simulink model "L150_Auto_Segments"  (R2026a)
settings: Solver=VariableStepAuto  StopTime=40.0
undefined symbols (not defined in the file): routeData, routeDirs, stopState
libraries: robotmobilelib x1, simulink x1
settings Model: Creator=hanjiatong  LastModifiedBy=hanjiatong

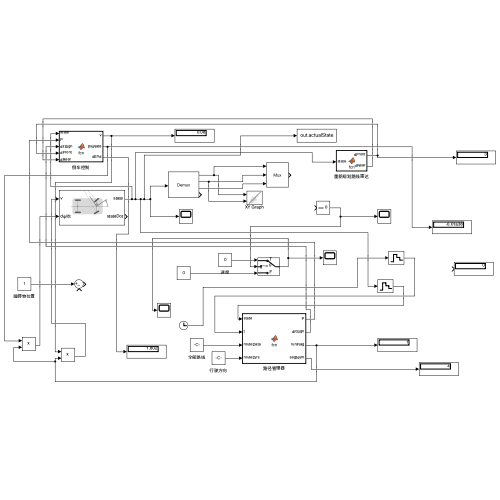
[thumbnail: Simulink's stored preview of the top-level diagram]
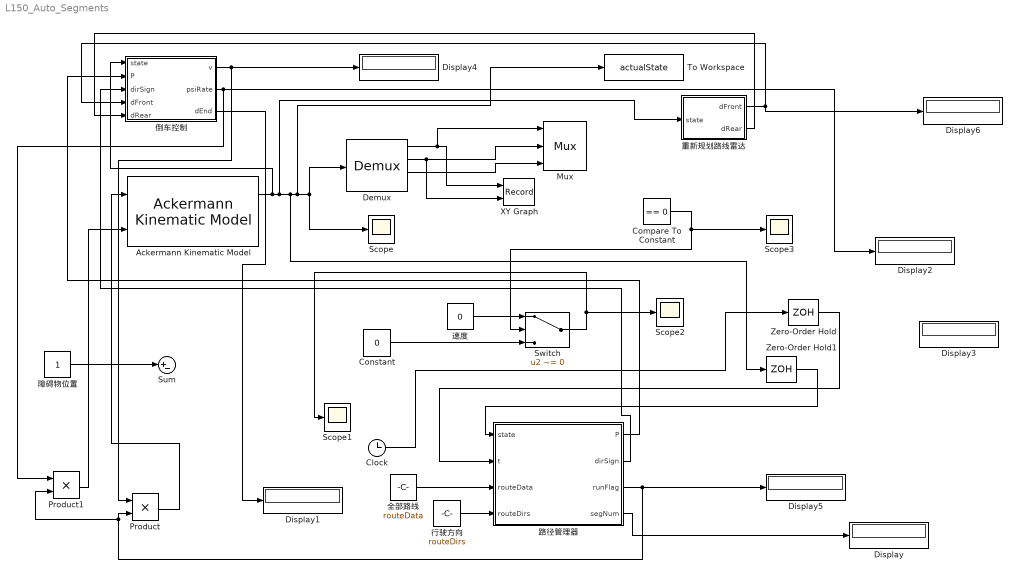
== system L150_Auto_Segments ==
  Ackermann Kinematic Model : robotmobilelib/Ackermann Kinematic Model  WheelBase=0.144  VehicleSpeedRange=[-inf inf]  MaxSteeringAngle=0.25  InitialState=stopState(:)  SimulateUsing=Interpreted execution
  Clock : Clock
  Compare To Constant : simulink/Logic and Bit Operations/Compare To Constant  relop===  const=0  OutDataTypeStr=boolean
  Constant : Constant  Value=0
  Demux : Demux
      settings: DisplayOption=none
  Display{,1..6} (7 alike) : Display
  Mux : Mux  Inputs=3
  Product : Product
  Product1 : Product
  Scope{,1..3} (4 alike) : Scope
      Scope settings: ActiveDisplayYMinimum=-0.19594221664657985  ActiveDisplayYMaximum=1.7514452129987257
      Scope1 settings: ActiveDisplayYMinimum=-1  ActiveDisplayYMaximum=1
      Scope2 settings: ActiveDisplayYMinimum=-0.018749999999999996  ActiveDisplayYMaximum=0.16874999999999998  DataLoggingVariableName=ScopeData2
      Scope3 settings: ActiveDisplayYMinimum=0.33124999999999571  ActiveDisplayYMaximum=1.018749999999998  DataLoggingVariableName=ScopeData3
  Sum : Sum  Inputs=|+-
  Switch : Switch  Criteria=u2 ~= 0  SaturateOnIntegerOverflow=off  InputSameDT=off
  To Workspace : ToWorkspace  VariableName=actualState  SaveFormat=Timeseries  SampleTime=-1
  XY Graph : Record  NumPorts=2.0  FileSettingsInternal="{\"entries\":[{\"content\":{\"excelSettings\":{\"content\":{},\"type\":\"Streamout.ExcelSettings\"},\"parquetSettings\":{\"content\":{},\"type\":\"Streamout.ParquetSettings\"}},\"type\":\"Streamout.FileSettingStorage\",\"uuid\":\"\"}],\"packageUris\":[\"http:\\/\\/schema.mathworks.com\\/mf0\\/streamout_blocks\\/R2020a\"],\"version\":\"1.0\"}"  FrameSettings=[0, 0]  Layout=[1 1]  SignalsInternal="{\"entries\":[{\"content\":{\"signals\":[{\"content\":{\"blockPath\":[],\"dimensions\":[1],\"domain\":\"\",\"lineColor\":\"#a2142f\",\"plots\":[ 1 ],\"port\":1,\"sid\":[\"\"],\"signalID\":1,\"signalName\":\"Demux:1\"},\"type\":\"RecordBlkView.Signal\",\"uuid\":\"\"},{\"content\":{\"blockPath\":[],\"dimensions\":[1],\"domain\":\"\",\"lineColor\":\"#139fff\",\"plots\":[ 1 ],\"port\":2,\"sid\":[\"\"],\"signalID\":2,\"signalName\":\"Demux:2\"},\"type\":\"RecordBlkView.Signal\",\"uuid\":\"\"}]},\"type\":\"RecordBlkView.InputSignals\",\"uuid\":\"\"}],\"packageUris\":[\"http:\\/\\/schema.mathworks.com\\/mf0\\/streamout_blocks\\/R2020a\"],\"version\":\"1.0\"}"  VisualizationBindings="{\"xyplotplugin\":{\"info\":[{\"series\":[{\"bindingParametersList\":[{\"parameter\":\"X-Axis\",\"signalID\":1,\"signalName\":\"Demux:1\"},{\"parameter\":\"Y-Axis\",\"signalID\":2,\"signalName\":\"Demux:2\"}],\"seriesID\":0}],\"subplotID\":1}]}}"  CompatibilityTag=XY
  Zero-Order Hold : ZeroOrderHold  SampleTime=0.05
  Zero-Order Hold1 : ZeroOrderHold  SampleTime=0.05
  倒车控制 : MATLAB Function  TreatAsAtomicUnit=on
  全部路线 : Constant  Value=routeData
  行驶方向 : Constant  Value=routeDirs
  路径管理器 : MATLAB Function  TreatAsAtomicUnit=on
  速度 : Constant  Value=0
  重新规划路线雷达 : MATLAB Function  TreatAsAtomicUnit=on
  障碍物位置 : Constant
  wires:
  Ackermann Kinematic Model/1 -> 倒车控制/1(state), 重新规划路线雷达/1(state), Zero-Order Hold1/1, Scope/1, Demux/1, To Workspace/1
  Demux/2 -> XY Graph/2, Mux/2
  障碍物位置/1 -> Sum/1
  Switch/1 -> Scope2/1, Scope1/1
  Compare To Constant/1 -> Scope3/1, Switch/2
  速度/1 -> Switch/1
  Constant/1 -> Switch/3
  Demux/1 -> Mux/1, XY Graph/1
  Demux/3 -> Mux/3
  重新规划路线雷达/1(dFront) -> 倒车控制/4(dFront), Display6/1
  重新规划路线雷达/2(dRear) -> 倒车控制/5(dRear)
  倒车控制/1(v) -> Product/1, Display4/1
  倒车控制/2(psiRate) -> Product1/1, Display2/1
  倒车控制/3(dEnd) -> Display1/1
  Clock/1 -> Zero-Order Hold/1
  全部路线/1 -> 路径管理器/3(routeData)
  路径管理器/1(P) -> 倒车控制/2(P)
  路径管理器/2(dirSign) -> 倒车控制/3(dirSign)
  行驶方向/1 -> 路径管理器/4(routeDirs)
  Zero-Order Hold/1 -> 路径管理器/2(t)
  Zero-Order Hold1/1 -> 路径管理器/1(state)
  路径管理器/3(runFlag) -> Product1/2, Product/2, Display5/1
  Product/1 -> Ackermann Kinematic Model/1
  Product1/1 -> Ackermann Kinematic Model/2
  路径管理器/4(segNum) -> Display/1

== matlab function L150_Auto_Segments/路径管理器 ==
  data: state input; P output; t input; routeData input; routeDirs input; dirSign output; runFlag output; segNum output

function [P,dirSign,runFlag,segNum] = ...
    fcn(state,t,routeData,routeDirs)

% 管理当前执行的路径段
% phase=0 行驶
% phase=1 停车等待换挡
% phase=2 全部完成

persistent k phase holdTime lastT

if isempty(k)
    k = 1;
    phase = 0;
    holdTime = 0;
    lastT = -1;
end

% 仿真重新开始时重置状态
if t < lastT - 1e-6
    k = 1;
    phase = 0;
    holdTime = 0;
end
lastT = t;

N = size(routeData,3);

% 读取当前路段
P = routeData(:,:,k);

% 当前路段终点距离
dEnd = hypot( ...
    P(end,1)-state(1), ...
    P(end,2)-state(2));

% 行驶状态
if phase == 0

    if dEnd <= 0.08

        if k == N
            % 所有路段完成
            phase = 2;
        else
            % 停车，准备换挡
            phase = 1;
            holdTime = t;
        end

    end

% 换挡等待状态
elseif phase == 1

    if t - holdTime >= 0.6
        k = k + 1;
        phase = 0;
    end

end

% 更新输出
P = routeData(:,:,k);
dirSign = routeDirs(k);
segNum = k;

dEnd = hypot( ...
    P(end,1)-state(1), ...
    P(end,2)-state(2));

% 只有行驶状态才允许运动
runFlag = double(phase == 0 && dEnd > 0.08);

end

== matlab function L150_Auto_Segments/重新规划路线雷达 ==
  data: state input; dFront output; dRear output

function [dFront,dRear] = fcn(state)

coder.extrinsic('l150ReplanLidar');

pose = [state(1),state(2),state(3)];

dFront = 3.0;
dRear = 3.0;

[dFront,dRear] = l150ReplanLidar(pose);

end

== matlab function L150_Auto_Segments/倒车控制 ==
  data: state input; v output; P input; dirSign input; dFront input; dRear input; psiRate output; dEnd output

function [v,psiRate,dEnd] = fcn( ...
    state,P,dirSign,dFront,dRear)

% state = [x y theta psi]
% P：当前要跟踪的一段路径
% dirSign：1前进，-1倒车

x = state(1);
y = state(2);
theta = state(3);
psi = state(4);

v = 0;
psiRate = 0;

% 当前路段终点距离
dEnd = hypot(P(end,1)-x,P(end,2)-y);

% 到达路段终点，停车
if dEnd <= 0.08
    return;
end

% 按行驶方向选择速度和安全雷达

% 仿真测试：按照规划方向行驶
% 暂时不使用雷达距离触发停车

if dirSign > 0
    v = 0.08;
else
    v = -0.06;
end


% 找出当前路段最近的路径点
n = size(P,1);
nearest = 1;
best = inf;

for i = 1:n
    d2 = (P(i,1)-x)^2 + (P(i,2)-y)^2;
    if d2 < best
        best = d2;
        nearest = i;
    end
end

% 沿路径向前寻找约0.25米的目标点
target = nearest;
travel = 0;

for i = nearest:n-1
    travel = travel + hypot( ...
        P(i+1,1)-P(i,1), ...
        P(i+1,2)-P(i,2));

    target = i+1;

    if travel >= 0.15
    break;
end
    
end

dx = P(target,1)-x;
dy = P(target,2)-y;

% 倒车时，运动方向与车头相反
moveHeading = theta;

if dirSign < 0
    moveHeading = theta + pi;
end

% 目标点在运动方向坐标系中的横向位置
yLocal = -sin(moveHeading)*dx ...
         + cos(moveHeading)*dy;

L2 = max(dx^2+dy^2,0.12^2);

% Pure Pursuit 几何曲率
kappa = 2*yLocal/L2;

% 倒车时需要反转转向曲率的符号
psiTarget = atan(0.144*dirSign*kappa);

% 限制转向角
psiTarget = max(-0.25,min(0.25,psiTarget));

% 计算前轮转向角速度
psiRate = 2*(psiTarget-psi);

% 限制转向角速度
psiRate = max(-0.35,min(0.35,psiRate));

end
